simulink model "controller_model"  (R2025b)
settings: Solver=ode4  StartTime=0.0  StopTime=tend  FixedStep=dt_rths  RelTol=1e-3
values from neighbouring files (symbols this model uses):
  dt_rths = 0.000244140625    [Plant.mat]    (also in RUN_vRTHS_demo_new.m)
  modified = 1    [RUN_vRTHS_demo_new.m]
  sat_limit_lower = -3.8    [F1_input_file.m]
  sat_limit_upper = +3.8    (= 3.8)    [F1_input_file.m]
undefined symbols (not defined in the file or in its folder): Acd, Apred, Bcd, Bpred, Ccd, Cpred, Dcd, digital_cntrlr, digital_cntrlr2, Dpred
settings Model: Creator=Sandra  LastModifiedBy=Victus
settings SolverCC: AlgebraicLoopSolver=TrustRegion
settings DataIOCC: SaveFormat=StructureWithTime  ReturnWorkspaceOutputs=off
settings OptimizationCC: LifeSpan=inf
settings DebuggingCC: InheritedTsInSrcMsg=none  UnconnectedInputMsg=warning  UnconnectedOutputMsg=warning  UnconnectedLineMsg=warning  SFExecutionAtInitializationDiag=none  ArithmeticOperatorsInVariantConditions=warning
settings HardwareCC: ProdBitPerSizeT=32.0  ProdBitPerPtrDiffT=32.0  ProdWordSize=32.0  ProdHWDeviceType=Specified
settings SFSimCC: SimUseLocalCustomCode=off  CustomCodeUndefinedFunction=UseInterfaceOnly
settings RTWCC: RTWUseLocalCustomCode=off  GPUComputeCapability=3.5
settings CodeAppCC: StateflowObjectComments=on

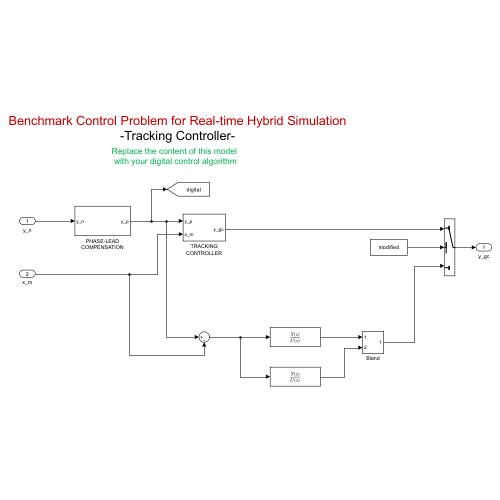
[thumbnail: Simulink's stored preview of the top-level diagram]
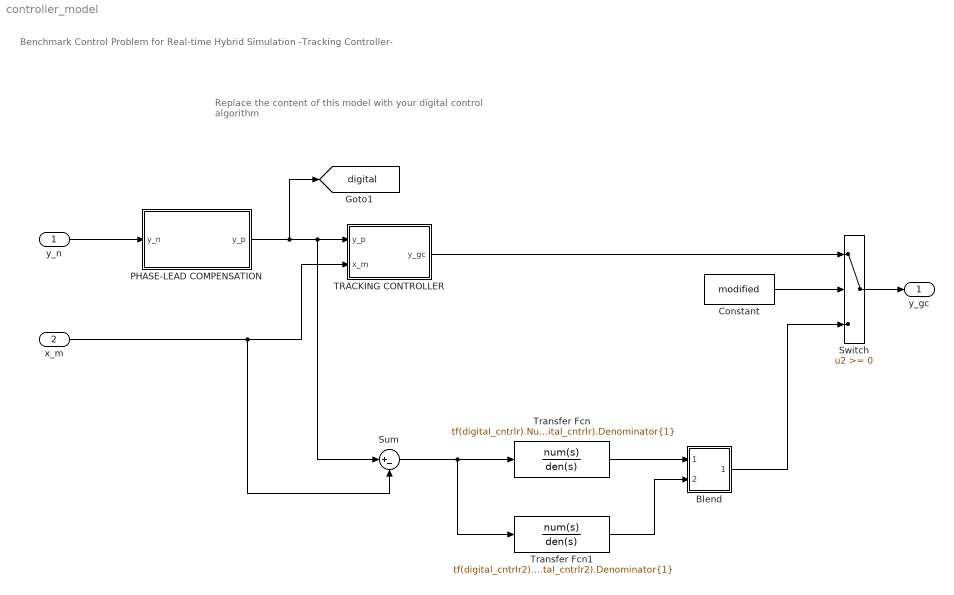
== system controller_model ==
  note: Benchmark Control Problem for Real-time Hybrid Simulation
      | -Tracking Controller-
  note: Replace the content of this model
      | with your digital control algorithm
  y_n : Inport
  x_m : Inport  Port=2
  Blend : Subsystem
  Constant : Constant  Value=modified
  PHASE-LEAD COMPENSATION : Subsystem
  Sum : Sum  Inputs=|+-
  Switch : Switch  SaturateOnIntegerOverflow=off  InputSameDT=off
  TRACKING CONTROLLER : Subsystem
  Transfer Fcn : TransferFcn  Numerator=tf(digital_cntrlr).Numerator{1}  Denominator=tf(digital_cntrlr).Denominator{1}
  Transfer Fcn1 : TransferFcn  Numerator=tf(digital_cntrlr2).Numerator{1}  Denominator=tf(digital_cntrlr2).Denominator{1}
  y_gc : Outport
  tag scope: digital=global
  wires:
  PHASE-LEAD COMPENSATION/1(y_p) -> [digital], Sum/1, TRACKING CONTROLLER/1(y_p)
  y_n/1 -> PHASE-LEAD COMPENSATION/1(y_n)
  x_m/1 -> Sum/2, TRACKING CONTROLLER/2(x_m)
  Sum/1 -> Transfer Fcn1/1, Transfer Fcn/1
  Transfer Fcn1/1 -> Blend/2(In2)
  Transfer Fcn/1 -> Blend/1(In1)
  Blend/1(Out1) -> Switch/3
  Switch/1 -> y_gc/1
  TRACKING CONTROLLER/1(y_gc) -> Switch/1
  Constant/1 -> Switch/2

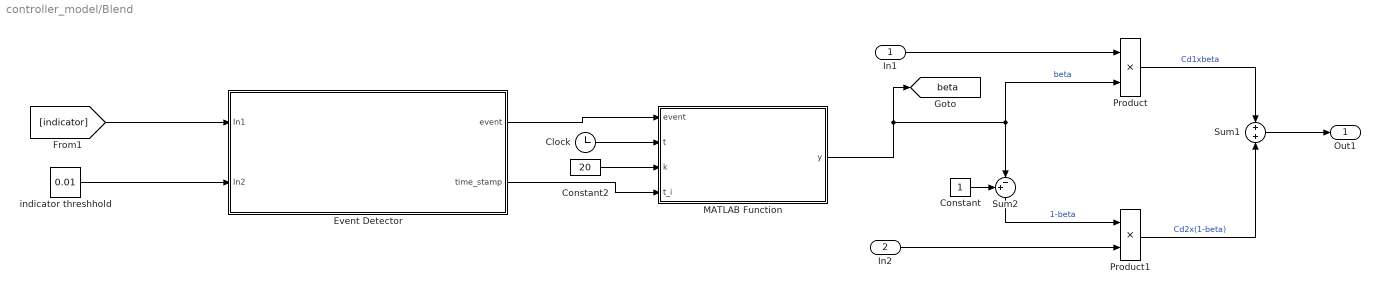
== system controller_model/Blend ==
  In1 : Inport
  In2 : Inport  Port=2
  Clock : Clock
  Constant : Constant
  Constant2 : Constant  Value=20
  Event Detector : Subsystem
  MATLAB Function : MATLAB Function  TreatAsAtomicUnit=on
  Product : Product
  Product1 : Product
  Sum1 : Sum
  Sum2 : Sum  Inputs=+-|
  indicator threshhold : Constant  Value=0.01
  Out1 : Outport
  tag scope: beta=global
  wires:
  Sum2/1 -> Product1/1  "1-beta"
  Sum1/1 -> Out1/1
  Product1/1 -> Sum1/2  "Cd2x(1-beta)"
  MATLAB Function/1(y) -> Product/2, Sum2/2, [beta]  "beta"
  Product/1 -> Sum1/1  "Cd1xbeta"
  Constant/1 -> Sum2/1
  In2/1 -> Product1/2
  In1/1 -> Product/1
  Event Detector/2(time_stamp) -> MATLAB Function/4(t_i)
  Constant2/1 -> MATLAB Function/3(k)
  [indicator] -> Event Detector/1(In1)
  indicator threshhold/1 -> Event Detector/2(In2)
  Event Detector/1(event) -> MATLAB Function/1(event)
  Clock/1 -> MATLAB Function/2(t)

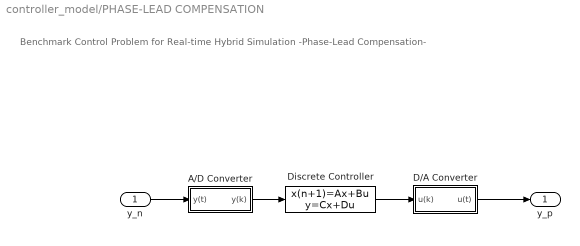
== system controller_model/PHASE-LEAD COMPENSATION ==
  note: Benchmark Control Problem for Real-time Hybrid Simulation
      | -Phase-Lead Compensation-
  y_n : Inport
  A/D Converter : Subsystem
  D/A Converter : Subsystem
  Discrete Controller : DiscreteStateSpace  A=Apred  B=Bpred  C=Cpred  D=Dpred  SampleTime=dt_rths
  y_p : Outport
  wires:
  Discrete Controller/1 -> D/A Converter/1(u(k))
  y_n/1 -> A/D Converter/1(y(t))
  A/D Converter/1(y(k)) -> Discrete Controller/1
  D/A Converter/1(u(t)) -> y_p/1

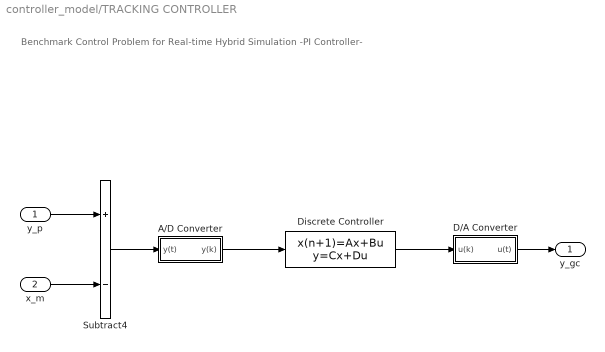
== system controller_model/TRACKING CONTROLLER ==
  note: Benchmark Control Problem for Real-time Hybrid Simulation
      | -PI Controller-
  y_p : Inport
  x_m : Inport  Port=2
  A/D Converter : Subsystem
  D/A Converter : Subsystem
  Discrete Controller : DiscreteStateSpace  A=Acd  B=Bcd  C=Ccd  D=Dcd  SampleTime=dt_rths
  Subtract4 : Sum  Inputs=+-
  y_gc : Outport
  wires:
  y_p/1 -> Subtract4/1
  Discrete Controller/1 -> D/A Converter/1(u(k))
  Subtract4/1 -> A/D Converter/1(y(t))
  x_m/1 -> Subtract4/2
  A/D Converter/1(y(k)) -> Discrete Controller/1
  D/A Converter/1(u(t)) -> y_gc/1

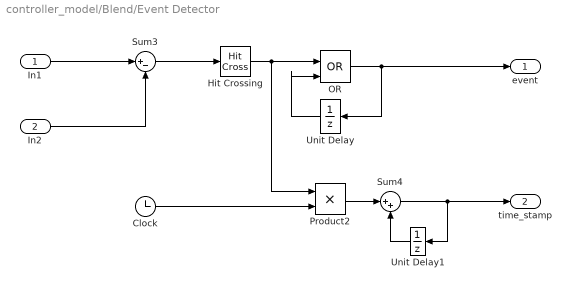
== system controller_model/Blend/Event Detector ==
  In1 : Inport
  In2 : Inport  Port=2
  Clock : Clock
  Hit Crossing : HitCross  HitCrossingDirection=falling
  OR : Logic  Operator=OR  IconShape=distinctive  AllPortsSameDT=off  OutDataTypeStr=boolean
  Product2 : Product
  Sum3 : Sum  Inputs=|+-
  Sum4 : Sum  Inputs=|++
  Unit Delay : UnitDelay  SampleTime=-1  HasFrameUpgradeWarning=on
  Unit Delay1 : UnitDelay  SampleTime=-1  HasFrameUpgradeWarning=on
  event : Outport
  time_stamp : Outport  Port=2
  wires:
  OR/1 -> event/1, Unit Delay/1
  Sum3/1 -> Hit Crossing/1
  Unit Delay/1 -> OR/2
  Sum4/1 -> time_stamp/1, Unit Delay1/1
  Unit Delay1/1 -> Sum4/2
  Hit Crossing/1 -> Product2/1, OR/1
  Clock/1 -> Product2/2
  Product2/1 -> Sum4/1
  In2/1 -> Sum3/2
  In1/1 -> Sum3/1

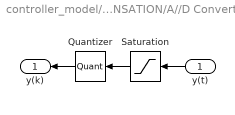
== system controller_model/PHASE-LEAD COMPENSATION/A//D Converter ==
  y(t) : Inport
  Quantizer : Quantizer  QuantizationInterval=quantize_int
  Saturation : Saturate  UpperLimit=sat_limit_upper  LowerLimit=sat_limit_lower
  y(k) : Outport
  wires:
  Saturation/1 -> Quantizer/1
  Quantizer/1 -> y(k)/1
  y(t)/1 -> Saturation/1

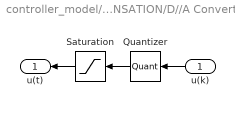
== system controller_model/PHASE-LEAD COMPENSATION/D//A Converter ==
  u(k) : Inport
  Quantizer : Quantizer  QuantizationInterval=quantize_int
  Saturation : Saturate  UpperLimit=sat_limit_upper  LowerLimit=sat_limit_lower
  u(t) : Outport
  wires:
  Saturation/1 -> u(t)/1
  Quantizer/1 -> Saturation/1
  u(k)/1 -> Quantizer/1

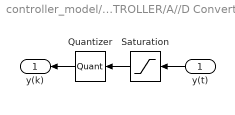
== system controller_model/TRACKING CONTROLLER/A//D Converter ==
  y(t) : Inport
  Quantizer : Quantizer  QuantizationInterval=quantize_int
  Saturation : Saturate  UpperLimit=sat_limit_upper  LowerLimit=sat_limit_lower
  y(k) : Outport
  wires:
  Saturation/1 -> Quantizer/1
  Quantizer/1 -> y(k)/1
  y(t)/1 -> Saturation/1

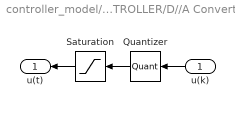
== system controller_model/TRACKING CONTROLLER/D//A Converter ==
  u(k) : Inport
  Quantizer : Quantizer  QuantizationInterval=quantize_int
  Saturation : Saturate  UpperLimit=sat_limit_upper  LowerLimit=sat_limit_lower
  u(t) : Outport
  wires:
  Saturation/1 -> u(t)/1
  Quantizer/1 -> Saturation/1
  u(k)/1 -> Quantizer/1

== matlab function controller_model/Blend/MATLAB Function ==
  data: event input; t input; y output; k input; t_i input
function y = beta_value(event, t, k, t_i)
%#codegen
% event : logical/boolean (1 -> force output to 0)
% t     : current sim time from a Clock block (scalar)
% k     : steepness
% t_s   : center time of the S-curve

    % Ensure scalar time (Clock already gives a scalar)
    tt = t;

    if ~event
        % If the event is active, force output to zero and exit.
        y = 1;
        return;
    end
    t_s = t_i + 5/k;  % pushes the steepest point to insure smooth transition (2.5/k is an emperical value)
    % Otherwise, logistic S-shaped value
    y = 1 - 1 / (1 + exp(-k * (tt - t_s)));
end
